simulink model "TB19_R2_Integrated_Shed"  (R2025a)
settings: Solver=FixedStepDiscrete  StartTime=0  StopTime=TB.t_end  FixedStep=TB.dt  RelTol=1e-3
InitFcn:
  | % 모델과 같은 폴더의 초기화 스크립트를 실행해 P(설계 파라미터)와 TB(시험 조건)를 만든다.
  | run(fullfile(fileparts(get_param(bdroot, 'FileName')), 'TB19_init.m'));
values from neighbouring files (symbols this model uses):
  TB = struct()    [TB19_init.m]    (also in run_TB19.m = evalin('base', 'TB'))
libraries: fl_lib x158, nesl_utility x67
(part 2 of 4)

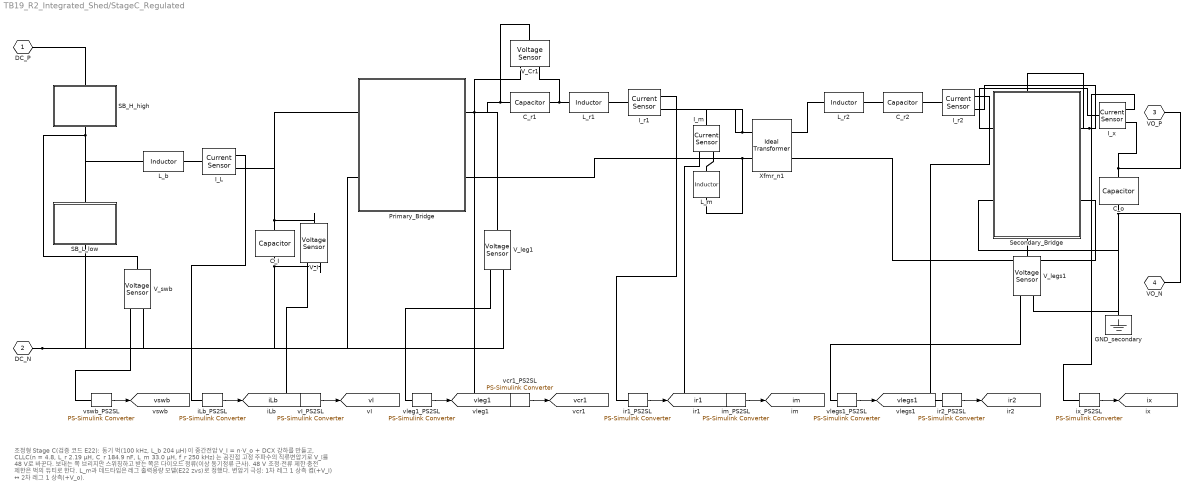
== system TB19_R2_Integrated_Shed/StageC_Regulated ==
  note: 조정형 Stage C(검증 코드 E22): 동기 벅(100 kHz, L_b 204 µH)이 중간전압 V_I = n·V_o + DCX 강하를 만들고,
      | CLLC(n = 4.8, L_r 2.19 µH, C_r 184.9 nF, L_m 33.0 µH, f_r 250 kHz)는 공진점 고정 주파수의 직류변압기로 V_I를 48 V로 바꾼다.
      | 보내는 쪽 브리지만 스위칭하고 받는 쪽은 다이오드 정류(이상 동기정류 근사). 48 V 조정·전류 제한·충전 제한은 벅의 듀티로 한다.
      | L_m과 데드타임은 레그 출력용량 모델(E22 zvs)로 정했다. 변압기 극성: 1차 레그 1 상측 켬(+V_I) ↔ 2차 레그 1 상측(+V_o).
  C_I : fl_lib/Electrical/Electrical Elements/Capacitor  c=TB.C.CI F  r=1e-6 Ohm  g=0 1/Ohm  i_specify=off  i_priority=None  i=0 A  i_nominal_specify=off  i_nominal_value=1  i_nominal_unit=A  v_specify=off  v_priority=None  v=0 V  v_nominal_specify=off  v_nominal_value=1  v_nominal_unit=V  vc_specify=on  vc_priority=High  vc=TB.x0(2) V  vc_nominal_specify=off  vc_nominal_value=1  vc_nominal_unit=V
  C_o : fl_lib/Electrical/Electrical Elements/Capacitor  c=TB.C.Co F  r=1e-6 Ohm  g=0 1/Ohm  i_specify=off  i_priority=None  i=0 A  i_nominal_specify=off  i_nominal_value=1  i_nominal_unit=A  v_specify=off  v_priority=None  v=0 V  v_nominal_specify=off  v_nominal_value=1  v_nominal_unit=V  vc_specify=on  vc_priority=High  vc=TB.x0(3) V  vc_nominal_specify=off  vc_nominal_value=1  vc_nominal_unit=V
  C_r1 : fl_lib/Electrical/Electrical Elements/Capacitor  c=TB.C.Cr1 F  r=1e-6 Ohm  g=0 1/Ohm  i_specify=off  i_priority=None  i=0 A  i_nominal_specify=off  i_nominal_value=1  i_nominal_unit=A  v_specify=off  v_priority=None  v=0 V  v_nominal_specify=off  v_nominal_value=1  v_nominal_unit=V  vc_specify=on  vc_priority=High  vc=0 V  vc_nominal_specify=off  vc_nominal_value=1  vc_nominal_unit=V
  C_r2 : fl_lib/Electrical/Electrical Elements/Capacitor  c=TB.C.Cr2 F  r=1e-6 Ohm  g=0 1/Ohm  i_specify=off  i_priority=None  i=0 A  i_nominal_specify=off  i_nominal_value=1  i_nominal_unit=A  v_specify=off  v_priority=None  v=0 V  v_nominal_specify=off  v_nominal_value=1  v_nominal_unit=V  vc_specify=on  vc_priority=High  vc=0 V  vc_nominal_specify=off  vc_nominal_value=1  vc_nominal_unit=V
  GND_secondary : fl_lib/Electrical/Electrical Elements/Electrical Reference
  I_L : fl_lib/Electrical/Electrical Sensors/Current Sensor
  I_m : fl_lib/Electrical/Electrical Sensors/Current Sensor
  I_r1 : fl_lib/Electrical/Electrical Sensors/Current Sensor
  I_r2 : fl_lib/Electrical/Electrical Sensors/Current Sensor
  I_x : fl_lib/Electrical/Electrical Sensors/Current Sensor
  L_b : fl_lib/Electrical/Electrical Elements/Inductor  l=TB.C.L H  r=TB.C.RL Ohm  g=1e-9 1/Ohm  i_specify=off  i_priority=None  i=0 A  i_nominal_specify=off  i_nominal_value=1  i_nominal_unit=A  v_specify=off  v_priority=None  v=0 V  v_nominal_specify=off  v_nominal_value=1  v_nominal_unit=V  i_L_specify=on  i_L_priority=High  i_L=TB.x0(1) A  i_L_nominal_specify=off  i_L_nominal_value=1  i_L_nominal_unit=A
  L_m : fl_lib/Electrical/Electrical Elements/Inductor  l=TB.C.Lm H  r=0 Ohm  g=1e-9 1/Ohm  i_specify=off  i_priority=None  i=0 A  i_nominal_specify=off  i_nominal_value=1  i_nominal_unit=A  v_specify=off  v_priority=None  v=0 V  v_nominal_specify=off  v_nominal_value=1  v_nominal_unit=V  i_L_specify=on  i_L_priority=High  i_L=0 A  i_L_nominal_specify=off  i_L_nominal_value=1  i_L_nominal_unit=A
  L_r1 : fl_lib/Electrical/Electrical Elements/Inductor  l=TB.C.Lr1 H  r=TB.C.Rw1 Ohm  g=1e-9 1/Ohm  i_specify=off  i_priority=None  i=0 A  i_nominal_specify=off  i_nominal_value=1  i_nominal_unit=A  v_specify=off  v_priority=None  v=0 V  v_nominal_specify=off  v_nominal_value=1  v_nominal_unit=V  i_L_specify=on  i_L_priority=High  i_L=0 A  i_L_nominal_specify=off  i_L_nominal_value=1  i_L_nominal_unit=A
  L_r2 : fl_lib/Electrical/Electrical Elements/Inductor  l=TB.C.Lr2 H  r=TB.C.Rw2 Ohm  g=1e-9 1/Ohm  i_specify=off  i_priority=None  i=0 A  i_nominal_specify=off  i_nominal_value=1  i_nominal_unit=A  v_specify=off  v_priority=None  v=0 V  v_nominal_specify=off  v_nominal_value=1  v_nominal_unit=V  i_L_specify=on  i_L_priority=High  i_L=0 A  i_L_nominal_specify=off  i_L_nominal_value=1  i_L_nominal_unit=A
  Primary_Bridge : Subsystem
  SB_H_high : Subsystem  mask(PRISM-Hub switch cell){Ron=TB.SB.Ron, Goff=TB.SB.Goff, Vf=TB.SB.Vf, Rd=TB.SB.Rd, Goffd=TB.SB.Goffd, Coss=TB.SB.Coss}
      mask prompts: Ron "도통 저항 R_on [Ohm]"; Goff "차단 컨덕턴스 G_off [S]"; Vf "다이오드 순방향 전압 Vf [V]"; Rd "다이오드 도통 저항 R_d [Ohm]"; Goffd "다이오드 차단 컨덕턴스 [S]"; Coss "출력용량 C_oss [F]"
      mask help: 전력 반도체 스위치 셀 SB_H. 게이트 태그 gS_BH.
      settings: AttributesFormatString=gate: gS_BH
      mask Display:
      | plot([0.50 0.50 ],[0.95 0.65 ],[0.50 0.74 ],[0.65 0.35 ],[0.50 0.50 ],[0.35 0.05 ]);
      | plot([0.50 0.20 0.20 ],[0.80 0.80 0.58 ],[0.20 0.20 0.50 ],[0.42 0.20 0.20 ]);
      | plot([0.20 0.10 0.30 0.20 ],[0.58 0.42 0.42 0.58 ],[0.10 0.30 ],[0.58 0.58 ]);
      | port_label('LConn',1,'D');
      | port_label('RConn',1,'S');
  SB_L_low : Subsystem  mask(PRISM-Hub switch cell){Ron=TB.SB.Ron, Goff=TB.SB.Goff, Vf=TB.SB.Vf, Rd=TB.SB.Rd, Goffd=TB.SB.Goffd, Coss=TB.SB.Coss}
      mask prompts: Ron "도통 저항 R_on [Ohm]"; Goff "차단 컨덕턴스 G_off [S]"; Vf "다이오드 순방향 전압 Vf [V]"; Rd "다이오드 도통 저항 R_d [Ohm]"; Goffd "다이오드 차단 컨덕턴스 [S]"; Coss "출력용량 C_oss [F]"
      mask help: 전력 반도체 스위치 셀 SB_L. 게이트 태그 gS_BL.
      settings: AttributesFormatString=gate: gS_BL
      mask Display:
      | plot([0.50 0.50 ],[0.95 0.65 ],[0.50 0.74 ],[0.65 0.35 ],[0.50 0.50 ],[0.35 0.05 ]);
      | plot([0.50 0.20 0.20 ],[0.80 0.80 0.58 ],[0.20 0.20 0.50 ],[0.42 0.20 0.20 ]);
      | plot([0.20 0.10 0.30 0.20 ],[0.58 0.42 0.42 0.58 ],[0.10 0.30 ],[0.58 0.58 ]);
      | port_label('LConn',1,'D');
      | port_label('RConn',1,'S');
  Secondary_Bridge : Subsystem
  V_Cr1 : fl_lib/Electrical/Electrical Sensors/Voltage Sensor
  V_I : fl_lib/Electrical/Electrical Sensors/Voltage Sensor
  V_leg1 : fl_lib/Electrical/Electrical Sensors/Voltage Sensor
  V_legs1 : fl_lib/Electrical/Electrical Sensors/Voltage Sensor
  V_swb : fl_lib/Electrical/Electrical Sensors/Voltage Sensor
  Xfmr_n1 : fl_lib/Electrical/Electrical Elements/Ideal Transformer  n=TB.C.n  i1_specify=off  i1_priority=None  i1=0 A  i1_nominal_specify=off  i1_nominal_value=1  i1_nominal_unit=A  v1_specify=off  v1_priority=None  v1=0 V  v1_nominal_specify=off  v1_nominal_value=1  v1_nominal_unit=V  i2_specify=off  i2_priority=None  i2=0 A  i2_nominal_specify=off  i2_nominal_value=1  i2_nominal_unit=A  v2_specify=off  v2_priority=None  v2=0 V  v2_nominal_specify=off  v2_nominal_value=1  v2_nominal_unit=V
  iLb_PS2SL : nesl_utility/PS-Simulink Converter  PhysicalDomain=network_engine_domain  SubClassName=ps_output  LeftPortType=input  RightPortType=output  PseudoPeriodic=off  Frequencies=[]  VectorFormat=inherit  Unit=inherit  AffineConversion=off
  im_PS2SL : nesl_utility/PS-Simulink Converter  PhysicalDomain=network_engine_domain  SubClassName=ps_output  LeftPortType=input  RightPortType=output  PseudoPeriodic=off  Frequencies=[]  VectorFormat=inherit  Unit=inherit  AffineConversion=off
  ir1_PS2SL : nesl_utility/PS-Simulink Converter  PhysicalDomain=network_engine_domain  SubClassName=ps_output  LeftPortType=input  RightPortType=output  PseudoPeriodic=off  Frequencies=[]  VectorFormat=inherit  Unit=inherit  AffineConversion=off
  ir2_PS2SL : nesl_utility/PS-Simulink Converter  PhysicalDomain=network_engine_domain  SubClassName=ps_output  LeftPortType=input  RightPortType=output  PseudoPeriodic=off  Frequencies=[]  VectorFormat=inherit  Unit=inherit  AffineConversion=off
  ix_PS2SL : nesl_utility/PS-Simulink Converter  PhysicalDomain=network_engine_domain  SubClassName=ps_output  LeftPortType=input  RightPortType=output  PseudoPeriodic=off  Frequencies=[]  VectorFormat=inherit  Unit=inherit  AffineConversion=off
  vI_PS2SL : nesl_utility/PS-Simulink Converter  PhysicalDomain=network_engine_domain  SubClassName=ps_output  LeftPortType=input  RightPortType=output  PseudoPeriodic=off  Frequencies=[]  VectorFormat=inherit  Unit=inherit  AffineConversion=off
  vcr1_PS2SL : nesl_utility/PS-Simulink Converter  PhysicalDomain=network_engine_domain  SubClassName=ps_output  LeftPortType=input  RightPortType=output  PseudoPeriodic=off  Frequencies=[]  VectorFormat=inherit  Unit=inherit  AffineConversion=off
  vleg1_PS2SL : nesl_utility/PS-Simulink Converter  PhysicalDomain=network_engine_domain  SubClassName=ps_output  LeftPortType=input  RightPortType=output  PseudoPeriodic=off  Frequencies=[]  VectorFormat=inherit  Unit=inherit  AffineConversion=off
  vlegs1_PS2SL : nesl_utility/PS-Simulink Converter  PhysicalDomain=network_engine_domain  SubClassName=ps_output  LeftPortType=input  RightPortType=output  PseudoPeriodic=off  Frequencies=[]  VectorFormat=inherit  Unit=inherit  AffineConversion=off
  vswb_PS2SL : nesl_utility/PS-Simulink Converter  PhysicalDomain=network_engine_domain  SubClassName=ps_output  LeftPortType=input  RightPortType=output  PseudoPeriodic=off  Frequencies=[]  VectorFormat=inherit  Unit=inherit  AffineConversion=off
  DC_P : PMIOPort  Side=Left
  DC_N : PMIOPort  Port=2  Side=Left
  VO_P : PMIOPort  Port=3  Side=Right
  VO_N : PMIOPort  Port=4  Side=Right
  tag scope: iLb=global, im=global, ir1=global, ir2=global, ix=global, vI=global, vcr1=global, vleg1=global, vlegs1=global, vswb=global
  wires:
  iLb_PS2SL/1 -> [iLb]
  vI_PS2SL/1 -> [vI]
  vswb_PS2SL/1 -> [vswb]
  ir1_PS2SL/1 -> [ir1]
  im_PS2SL/1 -> [im]
  ir2_PS2SL/1 -> [ir2]
  ix_PS2SL/1 -> [ix]
  vcr1_PS2SL/1 -> [vcr1]
  vleg1_PS2SL/1 -> [vleg1]
  vlegs1_PS2SL/1 -> [vlegs1]
  connections:
  SB_H_high/LConn1 -- DC_P/RConn1
  SB_L_low/LConn1 -- SB_H_high/RConn1 -- L_b/LConn1 -- V_swb/LConn1
  SB_L_low/RConn1 -- C_I/RConn1 -- V_I/RConn2 -- V_swb/RConn2 -- Primary_Bridge/LConn2 -- DC_N/RConn1 -- V_leg1/RConn2
  L_b/RConn1 -- I_L/LConn1
  I_L/RConn2 -- V_I/LConn1 -- C_I/LConn1 -- Primary_Bridge/LConn1
  C_r1/LConn1 -- Primary_Bridge/RConn1 -- V_leg1/LConn1 -- V_Cr1/LConn1
  L_r1/LConn1 -- C_r1/RConn1 -- V_Cr1/RConn2
  L_r1/RConn1 -- I_r1/LConn1
  Xfmr_n1/LConn1 -- I_r1/RConn2 -- I_m/LConn1
  Primary_Bridge/RConn2 -- Xfmr_n1/LConn2 -- L_m/RConn1
  I_m/RConn2 -- L_m/LConn1
  Xfmr_n1/RConn1 -- L_r2/LConn1
  L_r2/RConn1 -- C_r2/LConn1
  C_r2/RConn1 -- I_r2/LConn1
  Secondary_Bridge/RConn1 -- I_r2/RConn2 -- V_legs1/LConn1
  Xfmr_n1/RConn2 -- Secondary_Bridge/RConn2
  Secondary_Bridge/LConn1 -- I_x/LConn1
  C_o/LConn1 -- I_x/RConn2 -- VO_P/RConn1
  Secondary_Bridge/LConn2 -- VO_N/RConn1 -- V_legs1/RConn2 -- C_o/RConn1 -- GND_secondary/LConn1
  I_L/RConn1 -- iLb_PS2SL/LConn1
  V_I/RConn1 -- vI_PS2SL/LConn1
  V_swb/RConn1 -- vswb_PS2SL/LConn1
  I_r1/RConn1 -- ir1_PS2SL/LConn1
  I_m/RConn1 -- im_PS2SL/LConn1
  I_r2/RConn1 -- ir2_PS2SL/LConn1
  I_x/RConn1 -- ix_PS2SL/LConn1
  V_Cr1/RConn1 -- vcr1_PS2SL/LConn1
  V_leg1/RConn1 -- vleg1_PS2SL/LConn1
  V_legs1/RConn1 -- vlegs1_PS2SL/LConn1

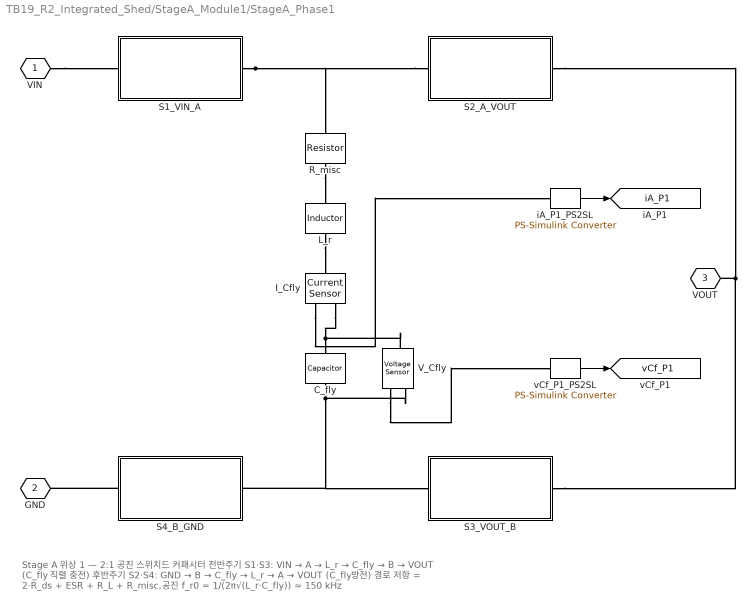
== system TB19_R2_Integrated_Shed/StageA_Module1/StageA_Phase1 ==
  note: Stage A 위상 1 — 2:1 공진 스위치드 커패시터
      | 전반주기 S1·S3: VIN → A → L_r → C_fly → B → VOUT (C_fly 직렬 충전)
      | 후반주기 S2·S4: GND → B → C_fly → L_r → A → VOUT (C_fly 방전)
      | 경로 저항 = 2·R_ds + ESR + R_L + R_misc, 공진 f_r0 = 1/(2π√(L_r·C_fly)) ≈ 150 kHz
  C_fly : fl_lib/Electrical/Electrical Elements/Capacitor  c=TB.A.Cfly F  r=TB.A.ESR Ohm  g=0 1/Ohm  i_specify=off  i_priority=None  i=0 A  i_nominal_specify=off  i_nominal_value=1  i_nominal_unit=A  v_specify=off  v_priority=None  v=0 V  v_nominal_specify=off  v_nominal_value=1  v_nominal_unit=V  vc_specify=on  vc_priority=High  vc=TB.A.vC0 V  vc_nominal_specify=off  vc_nominal_value=1  vc_nominal_unit=V
  I_Cfly : fl_lib/Electrical/Electrical Sensors/Current Sensor
  L_r : fl_lib/Electrical/Electrical Elements/Inductor  l=TB.A.Lr H  r=TB.A.RL Ohm  g=1e-9 1/Ohm  i_specify=off  i_priority=None  i=0 A  i_nominal_specify=off  i_nominal_value=1  i_nominal_unit=A  v_specify=off  v_priority=None  v=0 V  v_nominal_specify=off  v_nominal_value=1  v_nominal_unit=V  i_L_specify=on  i_L_priority=High  i_L=0 A  i_L_nominal_specify=off  i_L_nominal_value=1  i_L_nominal_unit=A
  R_misc : fl_lib/Electrical/Electrical Elements/Resistor  R=TB.A.Rmisc Ohm  i_specify=off  i_priority=None  i=0 A  i_nominal_specify=off  i_nominal_value=1  i_nominal_unit=A  v_specify=off  v_priority=None  v=0 V  v_nominal_specify=off  v_nominal_value=1  v_nominal_unit=V
  S1_VIN_A : Subsystem  mask(PRISM-Hub switch cell){Ron=TB.A.Rds, Goff=TB.A.Goff, Vf=TB.A.Vf, Rd=TB.A.Rd, Goffd=TB.A.Goffd}
      mask prompts: Ron "도통 저항 R_on [Ohm]"; Goff "차단 컨덕턴스 G_off [S]"; Vf "다이오드 순방향 전압 Vf [V]"; Rd "다이오드 도통 저항 R_d [Ohm]"; Goffd "다이오드 차단 컨덕턴스 [S]"
      mask help: 전력 반도체 스위치 셀 S1. 게이트 태그 gA_P1_S1.
      settings: AttributesFormatString=gate: gA_P1_S1
      mask Display:
      | plot([0.05 0.35 ],[0.50 0.50 ],[0.35 0.65 ],[0.50 0.74 ],[0.65 0.95 ],[0.50 0.50 ]);
      | plot([0.20 0.20 0.42 ],[0.50 0.20 0.20 ],[0.58 0.80 0.80 ],[0.20 0.20 0.50 ]);
      | plot([0.42 0.58 0.58 0.42 ],[0.20 0.10 0.30 0.20 ],[0.42 0.42 ],[0.10 0.30 ]);
      | text(0.5,0.80,'S1','horizontalAlignment','center','texmode','off');
      | port_label('LConn',1,'D');
      | port_label('RConn',1,'S');
  S2_A_VOUT : Subsystem  mask(PRISM-Hub switch cell){Ron=TB.A.Rds, Goff=TB.A.Goff, Vf=TB.A.Vf, Rd=TB.A.Rd, Goffd=TB.A.Goffd}
      mask prompts: Ron "도통 저항 R_on [Ohm]"; Goff "차단 컨덕턴스 G_off [S]"; Vf "다이오드 순방향 전압 Vf [V]"; Rd "다이오드 도통 저항 R_d [Ohm]"; Goffd "다이오드 차단 컨덕턴스 [S]"
      mask help: 전력 반도체 스위치 셀 S2. 게이트 태그 gA_P1_S2.
      settings: AttributesFormatString=gate: gA_P1_S2
      mask Display:
      | plot([0.05 0.35 ],[0.50 0.50 ],[0.35 0.65 ],[0.50 0.74 ],[0.65 0.95 ],[0.50 0.50 ]);
      | plot([0.20 0.20 0.42 ],[0.50 0.20 0.20 ],[0.58 0.80 0.80 ],[0.20 0.20 0.50 ]);
      | plot([0.42 0.58 0.58 0.42 ],[0.20 0.10 0.30 0.20 ],[0.42 0.42 ],[0.10 0.30 ]);
      | text(0.5,0.80,'S2','horizontalAlignment','center','texmode','off');
      | port_label('LConn',1,'D');
      | port_label('RConn',1,'S');
  S3_VOUT_B : Subsystem  mask(PRISM-Hub switch cell){Ron=TB.A.Rds, Goff=TB.A.Goff, Vf=TB.A.Vf, Rd=TB.A.Rd, Goffd=TB.A.Goffd}
      mask prompts: Ron "도통 저항 R_on [Ohm]"; Goff "차단 컨덕턴스 G_off [S]"; Vf "다이오드 순방향 전압 Vf [V]"; Rd "다이오드 도통 저항 R_d [Ohm]"; Goffd "다이오드 차단 컨덕턴스 [S]"
      mask help: 전력 반도체 스위치 셀 S3. 게이트 태그 gA_P1_S3.
      settings: AttributesFormatString=gate: gA_P1_S3
      mask Display:
      | plot([0.95 0.65 ],[0.50 0.50 ],[0.65 0.35 ],[0.50 0.74 ],[0.35 0.05 ],[0.50 0.50 ]);
      | plot([0.80 0.80 0.58 ],[0.50 0.20 0.20 ],[0.42 0.20 0.20 ],[0.20 0.20 0.50 ]);
      | plot([0.58 0.42 0.42 0.58 ],[0.20 0.10 0.30 0.20 ],[0.58 0.58 ],[0.10 0.30 ]);
      | text(0.5,0.80,'S3','horizontalAlignment','center','texmode','off');
      | port_label('LConn',1,'D');
      | port_label('RConn',1,'S');
  S4_B_GND : Subsystem  mask(PRISM-Hub switch cell){Ron=TB.A.Rds, Goff=TB.A.Goff, Vf=TB.A.Vf, Rd=TB.A.Rd, Goffd=TB.A.Goffd}
      mask prompts: Ron "도통 저항 R_on [Ohm]"; Goff "차단 컨덕턴스 G_off [S]"; Vf "다이오드 순방향 전압 Vf [V]"; Rd "다이오드 도통 저항 R_d [Ohm]"; Goffd "다이오드 차단 컨덕턴스 [S]"
      mask help: 전력 반도체 스위치 셀 S4. 게이트 태그 gA_P1_S4.
      settings: AttributesFormatString=gate: gA_P1_S4
      mask Display:
      | plot([0.95 0.65 ],[0.50 0.50 ],[0.65 0.35 ],[0.50 0.74 ],[0.35 0.05 ],[0.50 0.50 ]);
      | plot([0.80 0.80 0.58 ],[0.50 0.20 0.20 ],[0.42 0.20 0.20 ],[0.20 0.20 0.50 ]);
      | plot([0.58 0.42 0.42 0.58 ],[0.20 0.10 0.30 0.20 ],[0.58 0.58 ],[0.10 0.30 ]);
      | text(0.5,0.80,'S4','horizontalAlignment','center','texmode','off');
      | port_label('LConn',1,'D');
      | port_label('RConn',1,'S');
  V_Cfly : fl_lib/Electrical/Electrical Sensors/Voltage Sensor
  iA_P1_PS2SL : nesl_utility/PS-Simulink Converter  PhysicalDomain=network_engine_domain  SubClassName=ps_output  LeftPortType=input  RightPortType=output  PseudoPeriodic=off  Frequencies=[]  VectorFormat=inherit  Unit=inherit  AffineConversion=off
  vCf_P1_PS2SL : nesl_utility/PS-Simulink Converter  PhysicalDomain=network_engine_domain  SubClassName=ps_output  LeftPortType=input  RightPortType=output  PseudoPeriodic=off  Frequencies=[]  VectorFormat=inherit  Unit=inherit  AffineConversion=off
  VIN : PMIOPort  Side=Left
  GND : PMIOPort  Port=2  Side=Left
  VOUT : PMIOPort  Port=3  Side=Right
  tag scope: iA_P1=global, vCf_P1=global
  wires:
  iA_P1_PS2SL/1 -> [iA_P1]
  vCf_P1_PS2SL/1 -> [vCf_P1]
  connections:
  VIN/RConn1 -- S1_VIN_A/LConn1
  S2_A_VOUT/LConn1 -- S1_VIN_A/RConn1 -- R_misc/LConn1
  R_misc/RConn1 -- L_r/LConn1
  L_r/RConn1 -- I_Cfly/LConn1
  C_fly/LConn1 -- I_Cfly/RConn2 -- V_Cfly/LConn1
  S4_B_GND/LConn1 -- C_fly/RConn1 -- S3_VOUT_B/RConn1 -- V_Cfly/RConn2
  S4_B_GND/RConn1 -- GND/RConn1
  VOUT/RConn1 -- S2_A_VOUT/RConn1 -- S3_VOUT_B/LConn1
  I_Cfly/RConn1 -- iA_P1_PS2SL/LConn1
  V_Cfly/RConn1 -- vCf_P1_PS2SL/LConn1

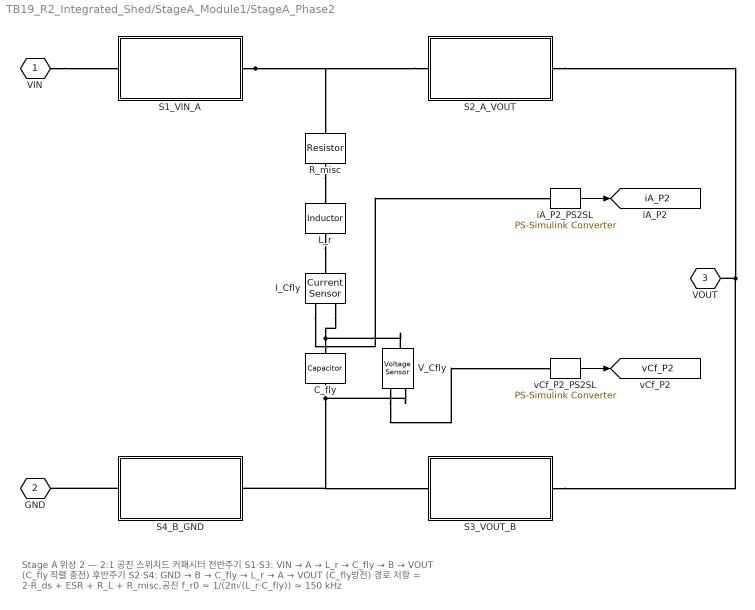
== system TB19_R2_Integrated_Shed/StageA_Module1/StageA_Phase2 ==
  note: Stage A 위상 2 — 2:1 공진 스위치드 커패시터
      | 전반주기 S1·S3: VIN → A → L_r → C_fly → B → VOUT (C_fly 직렬 충전)
      | 후반주기 S2·S4: GND → B → C_fly → L_r → A → VOUT (C_fly 방전)
      | 경로 저항 = 2·R_ds + ESR + R_L + R_misc, 공진 f_r0 = 1/(2π√(L_r·C_fly)) ≈ 150 kHz
  C_fly : fl_lib/Electrical/Electrical Elements/Capacitor  c=TB.A.Cfly F  r=TB.A.ESR Ohm  g=0 1/Ohm  i_specify=off  i_priority=None  i=0 A  i_nominal_specify=off  i_nominal_value=1  i_nominal_unit=A  v_specify=off  v_priority=None  v=0 V  v_nominal_specify=off  v_nominal_value=1  v_nominal_unit=V  vc_specify=on  vc_priority=High  vc=TB.A.vC0 V  vc_nominal_specify=off  vc_nominal_value=1  vc_nominal_unit=V
  I_Cfly : fl_lib/Electrical/Electrical Sensors/Current Sensor
  L_r : fl_lib/Electrical/Electrical Elements/Inductor  l=TB.A.Lr H  r=TB.A.RL Ohm  g=1e-9 1/Ohm  i_specify=off  i_priority=None  i=0 A  i_nominal_specify=off  i_nominal_value=1  i_nominal_unit=A  v_specify=off  v_priority=None  v=0 V  v_nominal_specify=off  v_nominal_value=1  v_nominal_unit=V  i_L_specify=on  i_L_priority=High  i_L=0 A  i_L_nominal_specify=off  i_L_nominal_value=1  i_L_nominal_unit=A
  R_misc : fl_lib/Electrical/Electrical Elements/Resistor  R=TB.A.Rmisc Ohm  i_specify=off  i_priority=None  i=0 A  i_nominal_specify=off  i_nominal_value=1  i_nominal_unit=A  v_specify=off  v_priority=None  v=0 V  v_nominal_specify=off  v_nominal_value=1  v_nominal_unit=V
  S1_VIN_A : Subsystem  mask(PRISM-Hub switch cell){Ron=TB.A.Rds, Goff=TB.A.Goff, Vf=TB.A.Vf, Rd=TB.A.Rd, Goffd=TB.A.Goffd}
      mask prompts: Ron "도통 저항 R_on [Ohm]"; Goff "차단 컨덕턴스 G_off [S]"; Vf "다이오드 순방향 전압 Vf [V]"; Rd "다이오드 도통 저항 R_d [Ohm]"; Goffd "다이오드 차단 컨덕턴스 [S]"
      mask help: 전력 반도체 스위치 셀 S1. 게이트 태그 gA_P2_S1.
      settings: AttributesFormatString=gate: gA_P2_S1
      mask Display:
      | plot([0.05 0.35 ],[0.50 0.50 ],[0.35 0.65 ],[0.50 0.74 ],[0.65 0.95 ],[0.50 0.50 ]);
      | plot([0.20 0.20 0.42 ],[0.50 0.20 0.20 ],[0.58 0.80 0.80 ],[0.20 0.20 0.50 ]);
      | plot([0.42 0.58 0.58 0.42 ],[0.20 0.10 0.30 0.20 ],[0.42 0.42 ],[0.10 0.30 ]);
      | text(0.5,0.80,'S1','horizontalAlignment','center','texmode','off');
      | port_label('LConn',1,'D');
      | port_label('RConn',1,'S');
  S2_A_VOUT : Subsystem  mask(PRISM-Hub switch cell){Ron=TB.A.Rds, Goff=TB.A.Goff, Vf=TB.A.Vf, Rd=TB.A.Rd, Goffd=TB.A.Goffd}
      mask prompts: Ron "도통 저항 R_on [Ohm]"; Goff "차단 컨덕턴스 G_off [S]"; Vf "다이오드 순방향 전압 Vf [V]"; Rd "다이오드 도통 저항 R_d [Ohm]"; Goffd "다이오드 차단 컨덕턴스 [S]"
      mask help: 전력 반도체 스위치 셀 S2. 게이트 태그 gA_P2_S2.
      settings: AttributesFormatString=gate: gA_P2_S2
      mask Display:
      | plot([0.05 0.35 ],[0.50 0.50 ],[0.35 0.65 ],[0.50 0.74 ],[0.65 0.95 ],[0.50 0.50 ]);
      | plot([0.20 0.20 0.42 ],[0.50 0.20 0.20 ],[0.58 0.80 0.80 ],[0.20 0.20 0.50 ]);
      | plot([0.42 0.58 0.58 0.42 ],[0.20 0.10 0.30 0.20 ],[0.42 0.42 ],[0.10 0.30 ]);
      | text(0.5,0.80,'S2','horizontalAlignment','center','texmode','off');
      | port_label('LConn',1,'D');
      | port_label('RConn',1,'S');
  S3_VOUT_B : Subsystem  mask(PRISM-Hub switch cell){Ron=TB.A.Rds, Goff=TB.A.Goff, Vf=TB.A.Vf, Rd=TB.A.Rd, Goffd=TB.A.Goffd}
      mask prompts: Ron "도통 저항 R_on [Ohm]"; Goff "차단 컨덕턴스 G_off [S]"; Vf "다이오드 순방향 전압 Vf [V]"; Rd "다이오드 도통 저항 R_d [Ohm]"; Goffd "다이오드 차단 컨덕턴스 [S]"
      mask help: 전력 반도체 스위치 셀 S3. 게이트 태그 gA_P2_S3.
      settings: AttributesFormatString=gate: gA_P2_S3
      mask Display:
      | plot([0.95 0.65 ],[0.50 0.50 ],[0.65 0.35 ],[0.50 0.74 ],[0.35 0.05 ],[0.50 0.50 ]);
      | plot([0.80 0.80 0.58 ],[0.50 0.20 0.20 ],[0.42 0.20 0.20 ],[0.20 0.20 0.50 ]);
      | plot([0.58 0.42 0.42 0.58 ],[0.20 0.10 0.30 0.20 ],[0.58 0.58 ],[0.10 0.30 ]);
      | text(0.5,0.80,'S3','horizontalAlignment','center','texmode','off');
      | port_label('LConn',1,'D');
      | port_label('RConn',1,'S');
  S4_B_GND : Subsystem  mask(PRISM-Hub switch cell){Ron=TB.A.Rds, Goff=TB.A.Goff, Vf=TB.A.Vf, Rd=TB.A.Rd, Goffd=TB.A.Goffd}
      mask prompts: Ron "도통 저항 R_on [Ohm]"; Goff "차단 컨덕턴스 G_off [S]"; Vf "다이오드 순방향 전압 Vf [V]"; Rd "다이오드 도통 저항 R_d [Ohm]"; Goffd "다이오드 차단 컨덕턴스 [S]"
      mask help: 전력 반도체 스위치 셀 S4. 게이트 태그 gA_P2_S4.
      settings: AttributesFormatString=gate: gA_P2_S4
      mask Display:
      | plot([0.95 0.65 ],[0.50 0.50 ],[0.65 0.35 ],[0.50 0.74 ],[0.35 0.05 ],[0.50 0.50 ]);
      | plot([0.80 0.80 0.58 ],[0.50 0.20 0.20 ],[0.42 0.20 0.20 ],[0.20 0.20 0.50 ]);
      | plot([0.58 0.42 0.42 0.58 ],[0.20 0.10 0.30 0.20 ],[0.58 0.58 ],[0.10 0.30 ]);
      | text(0.5,0.80,'S4','horizontalAlignment','center','texmode','off');
      | port_label('LConn',1,'D');
      | port_label('RConn',1,'S');
  V_Cfly : fl_lib/Electrical/Electrical Sensors/Voltage Sensor
  iA_P2_PS2SL : nesl_utility/PS-Simulink Converter  PhysicalDomain=network_engine_domain  SubClassName=ps_output  LeftPortType=input  RightPortType=output  PseudoPeriodic=off  Frequencies=[]  VectorFormat=inherit  Unit=inherit  AffineConversion=off
  vCf_P2_PS2SL : nesl_utility/PS-Simulink Converter  PhysicalDomain=network_engine_domain  SubClassName=ps_output  LeftPortType=input  RightPortType=output  PseudoPeriodic=off  Frequencies=[]  VectorFormat=inherit  Unit=inherit  AffineConversion=off
  VIN : PMIOPort  Side=Left
  GND : PMIOPort  Port=2  Side=Left
  VOUT : PMIOPort  Port=3  Side=Right
  tag scope: iA_P2=global, vCf_P2=global
  wires:
  iA_P2_PS2SL/1 -> [iA_P2]
  vCf_P2_PS2SL/1 -> [vCf_P2]
  connections:
  VIN/RConn1 -- S1_VIN_A/LConn1
  S2_A_VOUT/LConn1 -- S1_VIN_A/RConn1 -- R_misc/LConn1
  R_misc/RConn1 -- L_r/LConn1
  L_r/RConn1 -- I_Cfly/LConn1
  C_fly/LConn1 -- I_Cfly/RConn2 -- V_Cfly/LConn1
  S4_B_GND/LConn1 -- C_fly/RConn1 -- S3_VOUT_B/RConn1 -- V_Cfly/RConn2
  S4_B_GND/RConn1 -- GND/RConn1
  VOUT/RConn1 -- S2_A_VOUT/RConn1 -- S3_VOUT_B/LConn1
  I_Cfly/RConn1 -- iA_P2_PS2SL/LConn1
  V_Cfly/RConn1 -- vCf_P2_PS2SL/LConn1

== system TB19_R2_Integrated_Shed/StageB_Regulator/DAB_Primary ==
  note: DAB 1차 풀브리지(400 V 버스 측): 50 % 구형파, 상태 +1 → P1·P4, −1 → P2·P3
  P1_leg1_high : Subsystem  mask(PRISM-Hub switch cell){Ron=TB.B.Ron, Goff=TB.B.Goff, Vf=TB.B.Vf, Rd=TB.B.Rd, Goffd=TB.B.Goffd, Coss=TB.B.Coss_dp}
      mask prompts: Ron "도통 저항 R_on [Ohm]"; Goff "차단 컨덕턴스 G_off [S]"; Vf "다이오드 순방향 전압 Vf [V]"; Rd "다이오드 도통 저항 R_d [Ohm]"; Goffd "다이오드 차단 컨덕턴스 [S]"; Coss "출력용량 C_oss [F]"
      mask help: 전력 반도체 스위치 셀 P1_leg1_high. 게이트 태그 gD_P1.
      settings: AttributesFormatString=gate: gD_P1
      mask Display:
      | plot([0.50 0.50 ],[0.95 0.65 ],[0.50 0.74 ],[0.65 0.35 ],[0.50 0.50 ],[0.35 0.05 ]);
      | plot([0.50 0.20 0.20 ],[0.80 0.80 0.58 ],[0.20 0.20 0.50 ],[0.42 0.20 0.20 ]);
      | plot([0.20 0.10 0.30 0.20 ],[0.58 0.42 0.42 0.58 ],[0.10 0.30 ],[0.58 0.58 ]);
      | port_label('LConn',1,'D');
      | port_label('RConn',1,'S');
  P2_leg1_low : Subsystem  mask(PRISM-Hub switch cell){Ron=TB.B.Ron, Goff=TB.B.Goff, Vf=TB.B.Vf, Rd=TB.B.Rd, Goffd=TB.B.Goffd, Coss=TB.B.Coss_dp}
      mask prompts: Ron "도통 저항 R_on [Ohm]"; Goff "차단 컨덕턴스 G_off [S]"; Vf "다이오드 순방향 전압 Vf [V]"; Rd "다이오드 도통 저항 R_d [Ohm]"; Goffd "다이오드 차단 컨덕턴스 [S]"; Coss "출력용량 C_oss [F]"
      mask help: 전력 반도체 스위치 셀 P2_leg1_low. 게이트 태그 gD_P2.
      settings: AttributesFormatString=gate: gD_P2
      mask Display:
      | plot([0.50 0.50 ],[0.95 0.65 ],[0.50 0.74 ],[0.65 0.35 ],[0.50 0.50 ],[0.35 0.05 ]);
      | plot([0.50 0.20 0.20 ],[0.80 0.80 0.58 ],[0.20 0.20 0.50 ],[0.42 0.20 0.20 ]);
      | plot([0.20 0.10 0.30 0.20 ],[0.58 0.42 0.42 0.58 ],[0.10 0.30 ],[0.58 0.58 ]);
      | port_label('LConn',1,'D');
      | port_label('RConn',1,'S');
  P3_leg2_high : Subsystem  mask(PRISM-Hub switch cell){Ron=TB.B.Ron, Goff=TB.B.Goff, Vf=TB.B.Vf, Rd=TB.B.Rd, Goffd=TB.B.Goffd, Coss=TB.B.Coss_dp}
      mask prompts: Ron "도통 저항 R_on [Ohm]"; Goff "차단 컨덕턴스 G_off [S]"; Vf "다이오드 순방향 전압 Vf [V]"; Rd "다이오드 도통 저항 R_d [Ohm]"; Goffd "다이오드 차단 컨덕턴스 [S]"; Coss "출력용량 C_oss [F]"
      mask help: 전력 반도체 스위치 셀 P3_leg2_high. 게이트 태그 gD_P3.
      settings: AttributesFormatString=gate: gD_P3
      mask Display:
      | plot([0.50 0.50 ],[0.95 0.65 ],[0.50 0.74 ],[0.65 0.35 ],[0.50 0.50 ],[0.35 0.05 ]);
      | plot([0.50 0.20 0.20 ],[0.80 0.80 0.58 ],[0.20 0.20 0.50 ],[0.42 0.20 0.20 ]);
      | plot([0.20 0.10 0.30 0.20 ],[0.58 0.42 0.42 0.58 ],[0.10 0.30 ],[0.58 0.58 ]);
      | port_label('LConn',1,'D');
      | port_label('RConn',1,'S');
  P4_leg2_low : Subsystem  mask(PRISM-Hub switch cell){Ron=TB.B.Ron, Goff=TB.B.Goff, Vf=TB.B.Vf, Rd=TB.B.Rd, Goffd=TB.B.Goffd, Coss=TB.B.Coss_dp}
      mask prompts: Ron "도통 저항 R_on [Ohm]"; Goff "차단 컨덕턴스 G_off [S]"; Vf "다이오드 순방향 전압 Vf [V]"; Rd "다이오드 도통 저항 R_d [Ohm]"; Goffd "다이오드 차단 컨덕턴스 [S]"; Coss "출력용량 C_oss [F]"
      mask help: 전력 반도체 스위치 셀 P4_leg2_low. 게이트 태그 gD_P4.
      settings: AttributesFormatString=gate: gD_P4
      mask Display:
      | plot([0.50 0.50 ],[0.95 0.65 ],[0.50 0.74 ],[0.65 0.35 ],[0.50 0.50 ],[0.35 0.05 ]);
      | plot([0.50 0.20 0.20 ],[0.80 0.80 0.58 ],[0.20 0.20 0.50 ],[0.42 0.20 0.20 ]);
      | plot([0.20 0.10 0.30 0.20 ],[0.58 0.42 0.42 0.58 ],[0.10 0.30 ],[0.58 0.58 ]);
      | port_label('LConn',1,'D');
      | port_label('RConn',1,'S');
  DC_P : PMIOPort  Side=Left
  DC_N : PMIOPort  Port=2  Side=Left
  AC1 : PMIOPort  Port=3  Side=Right
  AC2 : PMIOPort  Port=4  Side=Right
  connections:
  P1_leg1_high/LConn1 -- DC_P/RConn1 -- P3_leg2_high/LConn1
  P2_leg1_low/LConn1 -- P1_leg1_high/RConn1 -- AC1/RConn1
  P4_leg2_low/LConn1 -- P3_leg2_high/RConn1 -- AC2/RConn1
  DC_N/RConn1 -- P2_leg1_low/RConn1 -- P4_leg2_low/RConn1

== system TB19_R2_Integrated_Shed/StageB_Regulator/DAB_Secondary ==
  note: DAB 2차 풀브리지(100 V 링크 측): 상태 +1 → S1·S4, −1 → S2·S3. 2차 에지 = 1차 에지 + δ
  S1_leg1_high : Subsystem  mask(PRISM-Hub switch cell){Ron=TB.B.Ron, Goff=TB.B.Goff, Vf=TB.B.Vf, Rd=TB.B.Rd, Goffd=TB.B.Goffd, Coss=TB.B.Coss_ds}
      mask prompts: Ron "도통 저항 R_on [Ohm]"; Goff "차단 컨덕턴스 G_off [S]"; Vf "다이오드 순방향 전압 Vf [V]"; Rd "다이오드 도통 저항 R_d [Ohm]"; Goffd "다이오드 차단 컨덕턴스 [S]"; Coss "출력용량 C_oss [F]"
      mask help: 전력 반도체 스위치 셀 S1_leg1_high. 게이트 태그 gD_S1.
      settings: AttributesFormatString=gate: gD_S1
      mask Display:
      | plot([0.50 0.50 ],[0.95 0.65 ],[0.50 0.74 ],[0.65 0.35 ],[0.50 0.50 ],[0.35 0.05 ]);
      | plot([0.50 0.20 0.20 ],[0.80 0.80 0.58 ],[0.20 0.20 0.50 ],[0.42 0.20 0.20 ]);
      | plot([0.20 0.10 0.30 0.20 ],[0.58 0.42 0.42 0.58 ],[0.10 0.30 ],[0.58 0.58 ]);
      | port_label('LConn',1,'D');
      | port_label('RConn',1,'S');
  S2_leg1_low : Subsystem  mask(PRISM-Hub switch cell){Ron=TB.B.Ron, Goff=TB.B.Goff, Vf=TB.B.Vf, Rd=TB.B.Rd, Goffd=TB.B.Goffd, Coss=TB.B.Coss_ds}
      mask prompts: Ron "도통 저항 R_on [Ohm]"; Goff "차단 컨덕턴스 G_off [S]"; Vf "다이오드 순방향 전압 Vf [V]"; Rd "다이오드 도통 저항 R_d [Ohm]"; Goffd "다이오드 차단 컨덕턴스 [S]"; Coss "출력용량 C_oss [F]"
      mask help: 전력 반도체 스위치 셀 S2_leg1_low. 게이트 태그 gD_S2.
      settings: AttributesFormatString=gate: gD_S2
      mask Display:
      | plot([0.50 0.50 ],[0.95 0.65 ],[0.50 0.74 ],[0.65 0.35 ],[0.50 0.50 ],[0.35 0.05 ]);
      | plot([0.50 0.20 0.20 ],[0.80 0.80 0.58 ],[0.20 0.20 0.50 ],[0.42 0.20 0.20 ]);
      | plot([0.20 0.10 0.30 0.20 ],[0.58 0.42 0.42 0.58 ],[0.10 0.30 ],[0.58 0.58 ]);
      | port_label('LConn',1,'D');
      | port_label('RConn',1,'S');
  S3_leg2_high : Subsystem  mask(PRISM-Hub switch cell){Ron=TB.B.Ron, Goff=TB.B.Goff, Vf=TB.B.Vf, Rd=TB.B.Rd, Goffd=TB.B.Goffd, Coss=TB.B.Coss_ds}
      mask prompts: Ron "도통 저항 R_on [Ohm]"; Goff "차단 컨덕턴스 G_off [S]"; Vf "다이오드 순방향 전압 Vf [V]"; Rd "다이오드 도통 저항 R_d [Ohm]"; Goffd "다이오드 차단 컨덕턴스 [S]"; Coss "출력용량 C_oss [F]"
      mask help: 전력 반도체 스위치 셀 S3_leg2_high. 게이트 태그 gD_S3.
      settings: AttributesFormatString=gate: gD_S3
      mask Display:
      | plot([0.50 0.50 ],[0.95 0.65 ],[0.50 0.74 ],[0.65 0.35 ],[0.50 0.50 ],[0.35 0.05 ]);
      | plot([0.50 0.20 0.20 ],[0.80 0.80 0.58 ],[0.20 0.20 0.50 ],[0.42 0.20 0.20 ]);
      | plot([0.20 0.10 0.30 0.20 ],[0.58 0.42 0.42 0.58 ],[0.10 0.30 ],[0.58 0.58 ]);
      | port_label('LConn',1,'D');
      | port_label('RConn',1,'S');
  S4_leg2_low : Subsystem  mask(PRISM-Hub switch cell){Ron=TB.B.Ron, Goff=TB.B.Goff, Vf=TB.B.Vf, Rd=TB.B.Rd, Goffd=TB.B.Goffd, Coss=TB.B.Coss_ds}
      mask prompts: Ron "도통 저항 R_on [Ohm]"; Goff "차단 컨덕턴스 G_off [S]"; Vf "다이오드 순방향 전압 Vf [V]"; Rd "다이오드 도통 저항 R_d [Ohm]"; Goffd "다이오드 차단 컨덕턴스 [S]"; Coss "출력용량 C_oss [F]"
      mask help: 전력 반도체 스위치 셀 S4_leg2_low. 게이트 태그 gD_S4.
      settings: AttributesFormatString=gate: gD_S4
      mask Display:
      | plot([0.50 0.50 ],[0.95 0.65 ],[0.50 0.74 ],[0.65 0.35 ],[0.50 0.50 ],[0.35 0.05 ]);
      | plot([0.50 0.20 0.20 ],[0.80 0.80 0.58 ],[0.20 0.20 0.50 ],[0.42 0.20 0.20 ]);
      | plot([0.20 0.10 0.30 0.20 ],[0.58 0.42 0.42 0.58 ],[0.10 0.30 ],[0.58 0.58 ]);
      | port_label('LConn',1,'D');
      | port_label('RConn',1,'S');
  DC_P : PMIOPort  Side=Left
  DC_N : PMIOPort  Port=2  Side=Left
  AC1 : PMIOPort  Port=3  Side=Right
  AC2 : PMIOPort  Port=4  Side=Right
  connections:
  S1_leg1_high/LConn1 -- DC_P/RConn1 -- S3_leg2_high/LConn1
  S2_leg1_low/LConn1 -- S1_leg1_high/RConn1 -- AC1/RConn1
  S4_leg2_low/LConn1 -- S3_leg2_high/RConn1 -- AC2/RConn1
  DC_N/RConn1 -- S2_leg1_low/RConn1 -- S4_leg2_low/RConn1

== system TB19_R2_Integrated_Shed/StageB_Regulator/HBridge ==
  note: Stage B H-브리지(4상한): 레그 A = QA_high/QA_low, 레그 B = QB_high/QB_low
      | 유니폴라 PWM 200 kHz, 데드타임 50 ns, 셀마다 C_oss 1 nF(레그 노드 등가 2 nF)
      | 출력 v_AB = v_A − v_B → L_h 필터 → 직렬 커패시터(직렬 포트)
  QA_high : Subsystem  mask(PRISM-Hub switch cell){Ron=TB.B.Ron, Goff=TB.B.Goff, Vf=TB.B.Vf, Rd=TB.B.Rd, Goffd=TB.B.Goffd, Coss=TB.B.Coss_h}
      mask prompts: Ron "도통 저항 R_on [Ohm]"; Goff "차단 컨덕턴스 G_off [S]"; Vf "다이오드 순방향 전압 Vf [V]"; Rd "다이오드 도통 저항 R_d [Ohm]"; Goffd "다이오드 차단 컨덕턴스 [S]"; Coss "출력용량 C_oss [F]"
      mask help: 전력 반도체 스위치 셀 QA_H. 게이트 태그 gB_AH.
      settings: AttributesFormatString=gate: gB_AH
      mask Display:
      | plot([0.50 0.50 ],[0.95 0.65 ],[0.50 0.74 ],[0.65 0.35 ],[0.50 0.50 ],[0.35 0.05 ]);
      | plot([0.50 0.20 0.20 ],[0.80 0.80 0.58 ],[0.20 0.20 0.50 ],[0.42 0.20 0.20 ]);
      | plot([0.20 0.10 0.30 0.20 ],[0.58 0.42 0.42 0.58 ],[0.10 0.30 ],[0.58 0.58 ]);
      | port_label('LConn',1,'D');
      | port_label('RConn',1,'S');
  QA_low : Subsystem  mask(PRISM-Hub switch cell){Ron=TB.B.Ron, Goff=TB.B.Goff, Vf=TB.B.Vf, Rd=TB.B.Rd, Goffd=TB.B.Goffd, Coss=TB.B.Coss_h}
      mask prompts: Ron "도통 저항 R_on [Ohm]"; Goff "차단 컨덕턴스 G_off [S]"; Vf "다이오드 순방향 전압 Vf [V]"; Rd "다이오드 도통 저항 R_d [Ohm]"; Goffd "다이오드 차단 컨덕턴스 [S]"; Coss "출력용량 C_oss [F]"
      mask help: 전력 반도체 스위치 셀 QA_L. 게이트 태그 gB_AL.
      settings: AttributesFormatString=gate: gB_AL
      mask Display:
      | plot([0.50 0.50 ],[0.95 0.65 ],[0.50 0.74 ],[0.65 0.35 ],[0.50 0.50 ],[0.35 0.05 ]);
      | plot([0.50 0.20 0.20 ],[0.80 0.80 0.58 ],[0.20 0.20 0.50 ],[0.42 0.20 0.20 ]);
      | plot([0.20 0.10 0.30 0.20 ],[0.58 0.42 0.42 0.58 ],[0.10 0.30 ],[0.58 0.58 ]);
      | port_label('LConn',1,'D');
      | port_label('RConn',1,'S');
  QB_high : Subsystem  mask(PRISM-Hub switch cell){Ron=TB.B.Ron, Goff=TB.B.Goff, Vf=TB.B.Vf, Rd=TB.B.Rd, Goffd=TB.B.Goffd, Coss=TB.B.Coss_h}
      mask prompts: Ron "도통 저항 R_on [Ohm]"; Goff "차단 컨덕턴스 G_off [S]"; Vf "다이오드 순방향 전압 Vf [V]"; Rd "다이오드 도통 저항 R_d [Ohm]"; Goffd "다이오드 차단 컨덕턴스 [S]"; Coss "출력용량 C_oss [F]"
      mask help: 전력 반도체 스위치 셀 QB_H. 게이트 태그 gB_BH.
      settings: AttributesFormatString=gate: gB_BH
      mask Display:
      | plot([0.50 0.50 ],[0.95 0.65 ],[0.50 0.74 ],[0.65 0.35 ],[0.50 0.50 ],[0.35 0.05 ]);
      | plot([0.50 0.20 0.20 ],[0.80 0.80 0.58 ],[0.20 0.20 0.50 ],[0.42 0.20 0.20 ]);
      | plot([0.20 0.10 0.30 0.20 ],[0.58 0.42 0.42 0.58 ],[0.10 0.30 ],[0.58 0.58 ]);
      | port_label('LConn',1,'D');
      | port_label('RConn',1,'S');
  QB_low : Subsystem  mask(PRISM-Hub switch cell){Ron=TB.B.Ron, Goff=TB.B.Goff, Vf=TB.B.Vf, Rd=TB.B.Rd, Goffd=TB.B.Goffd, Coss=TB.B.Coss_h}
      mask prompts: Ron "도통 저항 R_on [Ohm]"; Goff "차단 컨덕턴스 G_off [S]"; Vf "다이오드 순방향 전압 Vf [V]"; Rd "다이오드 도통 저항 R_d [Ohm]"; Goffd "다이오드 차단 컨덕턴스 [S]"; Coss "출력용량 C_oss [F]"
      mask help: 전력 반도체 스위치 셀 QB_L. 게이트 태그 gB_BL.
      settings: AttributesFormatString=gate: gB_BL
      mask Display:
      | plot([0.50 0.50 ],[0.95 0.65 ],[0.50 0.74 ],[0.65 0.35 ],[0.50 0.50 ],[0.35 0.05 ]);
      | plot([0.50 0.20 0.20 ],[0.80 0.80 0.58 ],[0.20 0.20 0.50 ],[0.42 0.20 0.20 ]);
      | plot([0.20 0.10 0.30 0.20 ],[0.58 0.42 0.42 0.58 ],[0.10 0.30 ],[0.58 0.58 ]);
      | port_label('LConn',1,'D');
      | port_label('RConn',1,'S');
  V_nodeA : fl_lib/Electrical/Electrical Sensors/Voltage Sensor
  vA_node_PS2SL : nesl_utility/PS-Simulink Converter  PhysicalDomain=network_engine_domain  SubClassName=ps_output  LeftPortType=input  RightPortType=output  PseudoPeriodic=off  Frequencies=[]  VectorFormat=inherit  Unit=inherit  AffineConversion=off
  LINK_P : PMIOPort  Side=Left
  LINK_N : PMIOPort  Port=2  Side=Left
  A : PMIOPort  Port=3  Side=Right
  B : PMIOPort  Port=4  Side=Right
  tag scope: vA_node=global
  wires:
  vA_node_PS2SL/1 -> [vA_node]
  connections:
  QA_high/LConn1 -- LINK_P/RConn1 -- QB_high/LConn1
  QA_high/RConn1 -- A/RConn1 -- QA_low/LConn1 -- V_nodeA/LConn1
  QB_low/LConn1 -- QB_high/RConn1 -- B/RConn1
  QA_low/RConn1 -- QB_low/RConn1 -- LINK_N/RConn1 -- V_nodeA/RConn2
  V_nodeA/RConn1 -- vA_node_PS2SL/LConn1

== system TB19_R2_Integrated_Shed/StageB_Regulator/S_BRK ==
  note: 스위치 셀: 이상 스위치(R_on, G_off) + 역병렬 바디 다이오드(Vf, R_d)
      | 게이트: 전역 태그 "gBrk" (> 0.5 이면 도통)
  D_body : fl_lib/Electrical/Electrical Elements/Diode  Vf=Vf V  Ron=Rd Ohm  Goff=Goffd 1/Ohm  i_specify=off  i_priority=None  i=0 A  i_nominal_specify=off  i_nominal_value=1  i_nominal_unit=A  v_specify=off  v_priority=None  v=0 V  v_nominal_specify=off  v_nominal_value=1  v_nominal_unit=V
  Gate_PS : nesl_utility/Simulink-PS Converter  PhysicalDomain=network_engine_domain  SubClassName=ps_input  LeftPortType=input  RightPortType=output  PseudoPeriodic=off  Frequencies=[]  NoiseDistribution=none  NoiseParameters=[]  Unit=1  AffineConversion=off  FilteringAndDerivatives=zero  SimscapeFilterOrder=1  InputFilterTimeConstant=0.001  UdotUserProvided=0
  SW : fl_lib/Electrical/Electrical Elements/Switch  R_closed=Ron Ohm  G_open=Goff 1/Ohm  Threshold=0.5  i_specify=off  i_priority=None  i=0 A  i_nominal_specify=off  i_nominal_value=1  i_nominal_unit=A  v_specify=off  v_priority=None  v=0 V  v_nominal_specify=off  v_nominal_value=1  v_nominal_unit=V
  D : PMIOPort  Side=Left
  S : PMIOPort  Port=2  Side=Right
  wires:
  [gBrk] -> Gate_PS/1
  connections:
  Gate_PS/RConn1 -- SW/RConn1
  SW/LConn1 -- D/RConn1 -- D_body/RConn1
  S/RConn1 -- SW/RConn2 -- D_body/LConn1

== system TB19_R2_Integrated_Shed/StageC_Regulated/Primary_Bridge ==
  note: Stage C 1차 풀브리지(650 V GaN 2병렬): 1차가 보낼 때 250 kHz 50 % 상보 + 데드타임 t_dp, 2차가 보낼 때는 꺼 두고 다이오드 정류(경부하 두 브리지 구동 모드에서는 같은 위상)
  Q1_leg1_high : Subsystem  mask(PRISM-Hub switch cell){Ron=TB.CP.Ron, Goff=TB.CP.Goff, Vf=TB.CP.Vf, Rd=TB.CP.Rd, Goffd=TB.CP.Goffd, Coss=TB.CP.Coss}
      mask prompts: Ron "도통 저항 R_on [Ohm]"; Goff "차단 컨덕턴스 G_off [S]"; Vf "다이오드 순방향 전압 Vf [V]"; Rd "다이오드 도통 저항 R_d [Ohm]"; Goffd "다이오드 차단 컨덕턴스 [S]"; Coss "출력용량 C_oss [F]"
      mask help: 전력 반도체 스위치 셀 Q1_leg1_high. 게이트 태그 gC_Q1.
      settings: AttributesFormatString=gate: gC_Q1
      mask Display:
      | plot([0.50 0.50 ],[0.95 0.65 ],[0.50 0.74 ],[0.65 0.35 ],[0.50 0.50 ],[0.35 0.05 ]);
      | plot([0.50 0.20 0.20 ],[0.80 0.80 0.58 ],[0.20 0.20 0.50 ],[0.42 0.20 0.20 ]);
      | plot([0.20 0.10 0.30 0.20 ],[0.58 0.42 0.42 0.58 ],[0.10 0.30 ],[0.58 0.58 ]);
      | port_label('LConn',1,'D');
      | port_label('RConn',1,'S');
  Q2_leg1_low : Subsystem  mask(PRISM-Hub switch cell){Ron=TB.CP.Ron, Goff=TB.CP.Goff, Vf=TB.CP.Vf, Rd=TB.CP.Rd, Goffd=TB.CP.Goffd, Coss=TB.CP.Coss}
      mask prompts: Ron "도통 저항 R_on [Ohm]"; Goff "차단 컨덕턴스 G_off [S]"; Vf "다이오드 순방향 전압 Vf [V]"; Rd "다이오드 도통 저항 R_d [Ohm]"; Goffd "다이오드 차단 컨덕턴스 [S]"; Coss "출력용량 C_oss [F]"
      mask help: 전력 반도체 스위치 셀 Q2_leg1_low. 게이트 태그 gC_Q2.
      settings: AttributesFormatString=gate: gC_Q2
      mask Display:
      | plot([0.50 0.50 ],[0.95 0.65 ],[0.50 0.74 ],[0.65 0.35 ],[0.50 0.50 ],[0.35 0.05 ]);
      | plot([0.50 0.20 0.20 ],[0.80 0.80 0.58 ],[0.20 0.20 0.50 ],[0.42 0.20 0.20 ]);
      | plot([0.20 0.10 0.30 0.20 ],[0.58 0.42 0.42 0.58 ],[0.10 0.30 ],[0.58 0.58 ]);
      | port_label('LConn',1,'D');
      | port_label('RConn',1,'S');
  Q3_leg2_high : Subsystem  mask(PRISM-Hub switch cell){Ron=TB.CP.Ron, Goff=TB.CP.Goff, Vf=TB.CP.Vf, Rd=TB.CP.Rd, Goffd=TB.CP.Goffd, Coss=TB.CP.Coss}
      mask prompts: Ron "도통 저항 R_on [Ohm]"; Goff "차단 컨덕턴스 G_off [S]"; Vf "다이오드 순방향 전압 Vf [V]"; Rd "다이오드 도통 저항 R_d [Ohm]"; Goffd "다이오드 차단 컨덕턴스 [S]"; Coss "출력용량 C_oss [F]"
      mask help: 전력 반도체 스위치 셀 Q3_leg2_high. 게이트 태그 gC_Q3.
      settings: AttributesFormatString=gate: gC_Q3
      mask Display:
      | plot([0.50 0.50 ],[0.95 0.65 ],[0.50 0.74 ],[0.65 0.35 ],[0.50 0.50 ],[0.35 0.05 ]);
      | plot([0.50 0.20 0.20 ],[0.80 0.80 0.58 ],[0.20 0.20 0.50 ],[0.42 0.20 0.20 ]);
      | plot([0.20 0.10 0.30 0.20 ],[0.58 0.42 0.42 0.58 ],[0.10 0.30 ],[0.58 0.58 ]);
      | port_label('LConn',1,'D');
      | port_label('RConn',1,'S');
  Q4_leg2_low : Subsystem  mask(PRISM-Hub switch cell){Ron=TB.CP.Ron, Goff=TB.CP.Goff, Vf=TB.CP.Vf, Rd=TB.CP.Rd, Goffd=TB.CP.Goffd, Coss=TB.CP.Coss}
      mask prompts: Ron "도통 저항 R_on [Ohm]"; Goff "차단 컨덕턴스 G_off [S]"; Vf "다이오드 순방향 전압 Vf [V]"; Rd "다이오드 도통 저항 R_d [Ohm]"; Goffd "다이오드 차단 컨덕턴스 [S]"; Coss "출력용량 C_oss [F]"
      mask help: 전력 반도체 스위치 셀 Q4_leg2_low. 게이트 태그 gC_Q4.
      settings: AttributesFormatString=gate: gC_Q4
      mask Display:
      | plot([0.50 0.50 ],[0.95 0.65 ],[0.50 0.74 ],[0.65 0.35 ],[0.50 0.50 ],[0.35 0.05 ]);
      | plot([0.50 0.20 0.20 ],[0.80 0.80 0.58 ],[0.20 0.20 0.50 ],[0.42 0.20 0.20 ]);
      | plot([0.20 0.10 0.30 0.20 ],[0.58 0.42 0.42 0.58 ],[0.10 0.30 ],[0.58 0.58 ]);
      | port_label('LConn',1,'D');
      | port_label('RConn',1,'S');
  DC_P : PMIOPort  Side=Left
  DC_N : PMIOPort  Port=2  Side=Left
  AC1 : PMIOPort  Port=3  Side=Right
  AC2 : PMIOPort  Port=4  Side=Right
  connections:
  Q1_leg1_high/LConn1 -- DC_P/RConn1 -- Q3_leg2_high/LConn1
  Q2_leg1_low/LConn1 -- Q1_leg1_high/RConn1 -- AC1/RConn1
  Q4_leg2_low/LConn1 -- Q3_leg2_high/RConn1 -- AC2/RConn1
  DC_N/RConn1 -- Q2_leg1_low/RConn1 -- Q4_leg2_low/RConn1

== system TB19_R2_Integrated_Shed/StageC_Regulated/SB_H_high ==
  note: 스위치 셀: 이상 스위치(R_on, G_off) + 역병렬 바디 다이오드(Vf, R_d) + 출력용량 C_oss
      | 게이트: 전역 태그 "gS_BH" (> 0.5 이면 도통)
  C_oss : fl_lib/Electrical/Electrical Elements/Capacitor  c=Coss F  r=1e-6 Ohm  g=0 1/Ohm  i_specify=off  i_priority=None  i=0 A  i_nominal_specify=off  i_nominal_value=1  i_nominal_unit=A  v_specify=off  v_priority=None  v=0 V  v_nominal_specify=off  v_nominal_value=1  v_nominal_unit=V  vc_specify=off  vc_priority=High  vc=0 V  vc_nominal_specify=off  vc_nominal_value=1  vc_nominal_unit=V
  D_body : fl_lib/Electrical/Electrical Elements/Diode  Vf=Vf V  Ron=Rd Ohm  Goff=Goffd 1/Ohm  i_specify=off  i_priority=None  i=0 A  i_nominal_specify=off  i_nominal_value=1  i_nominal_unit=A  v_specify=off  v_priority=None  v=0 V  v_nominal_specify=off  v_nominal_value=1  v_nominal_unit=V
  Gate_PS : nesl_utility/Simulink-PS Converter  PhysicalDomain=network_engine_domain  SubClassName=ps_input  LeftPortType=input  RightPortType=output  PseudoPeriodic=off  Frequencies=[]  NoiseDistribution=none  NoiseParameters=[]  Unit=1  AffineConversion=off  FilteringAndDerivatives=zero  SimscapeFilterOrder=1  InputFilterTimeConstant=0.001  UdotUserProvided=0
  SW : fl_lib/Electrical/Electrical Elements/Switch  R_closed=Ron Ohm  G_open=Goff 1/Ohm  Threshold=0.5  i_specify=off  i_priority=None  i=0 A  i_nominal_specify=off  i_nominal_value=1  i_nominal_unit=A  v_specify=off  v_priority=None  v=0 V  v_nominal_specify=off  v_nominal_value=1  v_nominal_unit=V
  D : PMIOPort  Side=Left
  S : PMIOPort  Port=2  Side=Right
  wires:
  [gS_BH] -> Gate_PS/1
  connections:
  Gate_PS/RConn1 -- SW/RConn1
  SW/LConn1 -- D/RConn1 -- D_body/RConn1 -- C_oss/LConn1
  SW/RConn2 -- D_body/LConn1 -- S/RConn1 -- C_oss/RConn1

== system TB19_R2_Integrated_Shed/StageC_Regulated/SB_L_low ==
  note: 스위치 셀: 이상 스위치(R_on, G_off) + 역병렬 바디 다이오드(Vf, R_d) + 출력용량 C_oss
      | 게이트: 전역 태그 "gS_BL" (> 0.5 이면 도통)
  C_oss : fl_lib/Electrical/Electrical Elements/Capacitor  c=Coss F  r=1e-6 Ohm  g=0 1/Ohm  i_specify=off  i_priority=None  i=0 A  i_nominal_specify=off  i_nominal_value=1  i_nominal_unit=A  v_specify=off  v_priority=None  v=0 V  v_nominal_specify=off  v_nominal_value=1  v_nominal_unit=V  vc_specify=off  vc_priority=High  vc=0 V  vc_nominal_specify=off  vc_nominal_value=1  vc_nominal_unit=V
  D_body : fl_lib/Electrical/Electrical Elements/Diode  Vf=Vf V  Ron=Rd Ohm  Goff=Goffd 1/Ohm  i_specify=off  i_priority=None  i=0 A  i_nominal_specify=off  i_nominal_value=1  i_nominal_unit=A  v_specify=off  v_priority=None  v=0 V  v_nominal_specify=off  v_nominal_value=1  v_nominal_unit=V
  Gate_PS : nesl_utility/Simulink-PS Converter  PhysicalDomain=network_engine_domain  SubClassName=ps_input  LeftPortType=input  RightPortType=output  PseudoPeriodic=off  Frequencies=[]  NoiseDistribution=none  NoiseParameters=[]  Unit=1  AffineConversion=off  FilteringAndDerivatives=zero  SimscapeFilterOrder=1  InputFilterTimeConstant=0.001  UdotUserProvided=0
  SW : fl_lib/Electrical/Electrical Elements/Switch  R_closed=Ron Ohm  G_open=Goff 1/Ohm  Threshold=0.5  i_specify=off  i_priority=None  i=0 A  i_nominal_specify=off  i_nominal_value=1  i_nominal_unit=A  v_specify=off  v_priority=None  v=0 V  v_nominal_specify=off  v_nominal_value=1  v_nominal_unit=V
  D : PMIOPort  Side=Left
  S : PMIOPort  Port=2  Side=Right
  wires:
  [gS_BL] -> Gate_PS/1
  connections:
  Gate_PS/RConn1 -- SW/RConn1
  SW/LConn1 -- D/RConn1 -- D_body/RConn1 -- C_oss/LConn1
  SW/RConn2 -- D_body/LConn1 -- S/RConn1 -- C_oss/RConn1

== system TB19_R2_Integrated_Shed/StageC_Regulated/Secondary_Bridge ==
  note: Stage C 2차 풀브리지(150 V GaN 2병렬): 1차가 보낼 때는 꺼 두고 다이오드 정류(이상 동기정류 근사), 2차가 보낼 때 250 kHz + 데드타임 t_ds
  S1_leg1_high : Subsystem  mask(PRISM-Hub switch cell){Ron=TB.CS.Ron, Goff=TB.CS.Goff, Vf=TB.CS.Vf, Rd=TB.CS.Rd, Goffd=TB.CS.Goffd, Coss=TB.CS.Coss}
      mask prompts: Ron "도통 저항 R_on [Ohm]"; Goff "차단 컨덕턴스 G_off [S]"; Vf "다이오드 순방향 전압 Vf [V]"; Rd "다이오드 도통 저항 R_d [Ohm]"; Goffd "다이오드 차단 컨덕턴스 [S]"; Coss "출력용량 C_oss [F]"
      mask help: 전력 반도체 스위치 셀 S1_leg1_high. 게이트 태그 gC_S1.
      settings: AttributesFormatString=gate: gC_S1
      mask Display:
      | plot([0.50 0.50 ],[0.95 0.65 ],[0.50 0.74 ],[0.65 0.35 ],[0.50 0.50 ],[0.35 0.05 ]);
      | plot([0.50 0.20 0.20 ],[0.80 0.80 0.58 ],[0.20 0.20 0.50 ],[0.42 0.20 0.20 ]);
      | plot([0.20 0.10 0.30 0.20 ],[0.58 0.42 0.42 0.58 ],[0.10 0.30 ],[0.58 0.58 ]);
      | port_label('LConn',1,'D');
      | port_label('RConn',1,'S');
  S2_leg1_low : Subsystem  mask(PRISM-Hub switch cell){Ron=TB.CS.Ron, Goff=TB.CS.Goff, Vf=TB.CS.Vf, Rd=TB.CS.Rd, Goffd=TB.CS.Goffd, Coss=TB.CS.Coss}
      mask prompts: Ron "도통 저항 R_on [Ohm]"; Goff "차단 컨덕턴스 G_off [S]"; Vf "다이오드 순방향 전압 Vf [V]"; Rd "다이오드 도통 저항 R_d [Ohm]"; Goffd "다이오드 차단 컨덕턴스 [S]"; Coss "출력용량 C_oss [F]"
      mask help: 전력 반도체 스위치 셀 S2_leg1_low. 게이트 태그 gC_S2.
      settings: AttributesFormatString=gate: gC_S2
      mask Display:
      | plot([0.50 0.50 ],[0.95 0.65 ],[0.50 0.74 ],[0.65 0.35 ],[0.50 0.50 ],[0.35 0.05 ]);
      | plot([0.50 0.20 0.20 ],[0.80 0.80 0.58 ],[0.20 0.20 0.50 ],[0.42 0.20 0.20 ]);
      | plot([0.20 0.10 0.30 0.20 ],[0.58 0.42 0.42 0.58 ],[0.10 0.30 ],[0.58 0.58 ]);
      | port_label('LConn',1,'D');
      | port_label('RConn',1,'S');
  S3_leg2_high : Subsystem  mask(PRISM-Hub switch cell){Ron=TB.CS.Ron, Goff=TB.CS.Goff, Vf=TB.CS.Vf, Rd=TB.CS.Rd, Goffd=TB.CS.Goffd, Coss=TB.CS.Coss}
      mask prompts: Ron "도통 저항 R_on [Ohm]"; Goff "차단 컨덕턴스 G_off [S]"; Vf "다이오드 순방향 전압 Vf [V]"; Rd "다이오드 도통 저항 R_d [Ohm]"; Goffd "다이오드 차단 컨덕턴스 [S]"; Coss "출력용량 C_oss [F]"
      mask help: 전력 반도체 스위치 셀 S3_leg2_high. 게이트 태그 gC_S3.
      settings: AttributesFormatString=gate: gC_S3
      mask Display:
      | plot([0.50 0.50 ],[0.95 0.65 ],[0.50 0.74 ],[0.65 0.35 ],[0.50 0.50 ],[0.35 0.05 ]);
      | plot([0.50 0.20 0.20 ],[0.80 0.80 0.58 ],[0.20 0.20 0.50 ],[0.42 0.20 0.20 ]);
      | plot([0.20 0.10 0.30 0.20 ],[0.58 0.42 0.42 0.58 ],[0.10 0.30 ],[0.58 0.58 ]);
      | port_label('LConn',1,'D');
      | port_label('RConn',1,'S');
  S4_leg2_low : Subsystem  mask(PRISM-Hub switch cell){Ron=TB.CS.Ron, Goff=TB.CS.Goff, Vf=TB.CS.Vf, Rd=TB.CS.Rd, Goffd=TB.CS.Goffd, Coss=TB.CS.Coss}
      mask prompts: Ron "도통 저항 R_on [Ohm]"; Goff "차단 컨덕턴스 G_off [S]"; Vf "다이오드 순방향 전압 Vf [V]"; Rd "다이오드 도통 저항 R_d [Ohm]"; Goffd "다이오드 차단 컨덕턴스 [S]"; Coss "출력용량 C_oss [F]"
      mask help: 전력 반도체 스위치 셀 S4_leg2_low. 게이트 태그 gC_S4.
      settings: AttributesFormatString=gate: gC_S4
      mask Display:
      | plot([0.50 0.50 ],[0.95 0.65 ],[0.50 0.74 ],[0.65 0.35 ],[0.50 0.50 ],[0.35 0.05 ]);
      | plot([0.50 0.20 0.20 ],[0.80 0.80 0.58 ],[0.20 0.20 0.50 ],[0.42 0.20 0.20 ]);
      | plot([0.20 0.10 0.30 0.20 ],[0.58 0.42 0.42 0.58 ],[0.10 0.30 ],[0.58 0.58 ]);
      | port_label('LConn',1,'D');
      | port_label('RConn',1,'S');
  DC_P : PMIOPort  Side=Left
  DC_N : PMIOPort  Port=2  Side=Left
  AC1 : PMIOPort  Port=3  Side=Right
  AC2 : PMIOPort  Port=4  Side=Right
  connections:
  S1_leg1_high/LConn1 -- DC_P/RConn1 -- S3_leg2_high/LConn1
  S2_leg1_low/LConn1 -- S1_leg1_high/RConn1 -- AC1/RConn1
  S4_leg2_low/LConn1 -- S3_leg2_high/RConn1 -- AC2/RConn1
  DC_N/RConn1 -- S2_leg1_low/RConn1 -- S4_leg2_low/RConn1

== system TB19_R2_Integrated_Shed/StageA_Module1/StageA_Phase1/S1_VIN_A ==
  note: 스위치 셀: 이상 스위치(R_on, G_off) + 역병렬 바디 다이오드(Vf, R_d)
      | 게이트: 전역 태그 "gA_P1_S1" (> 0.5 이면 도통)
  D_body : fl_lib/Electrical/Electrical Elements/Diode  Vf=Vf V  Ron=Rd Ohm  Goff=Goffd 1/Ohm  i_specify=off  i_priority=None  i=0 A  i_nominal_specify=off  i_nominal_value=1  i_nominal_unit=A  v_specify=off  v_priority=None  v=0 V  v_nominal_specify=off  v_nominal_value=1  v_nominal_unit=V
  Gate_PS : nesl_utility/Simulink-PS Converter  PhysicalDomain=network_engine_domain  SubClassName=ps_input  LeftPortType=input  RightPortType=output  PseudoPeriodic=off  Frequencies=[]  NoiseDistribution=none  NoiseParameters=[]  Unit=1  AffineConversion=off  FilteringAndDerivatives=zero  SimscapeFilterOrder=1  InputFilterTimeConstant=0.001  UdotUserProvided=0
  SW : fl_lib/Electrical/Electrical Elements/Switch  R_closed=Ron Ohm  G_open=Goff 1/Ohm  Threshold=0.5  i_specify=off  i_priority=None  i=0 A  i_nominal_specify=off  i_nominal_value=1  i_nominal_unit=A  v_specify=off  v_priority=None  v=0 V  v_nominal_specify=off  v_nominal_value=1  v_nominal_unit=V
  D : PMIOPort  Side=Left
  S : PMIOPort  Port=2  Side=Right
  wires:
  [gA_P1_S1] -> Gate_PS/1
  connections:
  Gate_PS/RConn1 -- SW/RConn1
  SW/LConn1 -- D/RConn1 -- D_body/RConn1
  S/RConn1 -- SW/RConn2 -- D_body/LConn1

== system TB19_R2_Integrated_Shed/StageA_Module1/StageA_Phase1/S2_A_VOUT ==
  note: 스위치 셀: 이상 스위치(R_on, G_off) + 역병렬 바디 다이오드(Vf, R_d)
      | 게이트: 전역 태그 "gA_P1_S2" (> 0.5 이면 도통)
  D_body : fl_lib/Electrical/Electrical Elements/Diode  Vf=Vf V  Ron=Rd Ohm  Goff=Goffd 1/Ohm  i_specify=off  i_priority=None  i=0 A  i_nominal_specify=off  i_nominal_value=1  i_nominal_unit=A  v_specify=off  v_priority=None  v=0 V  v_nominal_specify=off  v_nominal_value=1  v_nominal_unit=V
  Gate_PS : nesl_utility/Simulink-PS Converter  PhysicalDomain=network_engine_domain  SubClassName=ps_input  LeftPortType=input  RightPortType=output  PseudoPeriodic=off  Frequencies=[]  NoiseDistribution=none  NoiseParameters=[]  Unit=1  AffineConversion=off  FilteringAndDerivatives=zero  SimscapeFilterOrder=1  InputFilterTimeConstant=0.001  UdotUserProvided=0
  SW : fl_lib/Electrical/Electrical Elements/Switch  R_closed=Ron Ohm  G_open=Goff 1/Ohm  Threshold=0.5  i_specify=off  i_priority=None  i=0 A  i_nominal_specify=off  i_nominal_value=1  i_nominal_unit=A  v_specify=off  v_priority=None  v=0 V  v_nominal_specify=off  v_nominal_value=1  v_nominal_unit=V
  D : PMIOPort  Side=Left
  S : PMIOPort  Port=2  Side=Right
  wires:
  [gA_P1_S2] -> Gate_PS/1
  connections:
  Gate_PS/RConn1 -- SW/RConn1
  SW/LConn1 -- D/RConn1 -- D_body/RConn1
  S/RConn1 -- SW/RConn2 -- D_body/LConn1
